simulink model "aerodynamic_model_V1_1_Coupling"  (R2025b)
settings: Solver=ode4  StartTime=0.0  StopTime=8  FixedStep=Ts  RelTol=1e-3
InitFcn:
  | % Run initial_main.m first to load Ad,As,Tq_prop,Tq_mass,...
values from neighbouring files (symbols this model uses):
  alpha_du0_v_tail_L = trim_aero_ic.v_tail_L.alpha_du0    [initial_main_V1_1.m]
  alpha_du0_v_tail_R = trim_aero_ic.v_tail_R.alpha_du0    [initial_main_V1_1.m]
  alpha_du0_wing_L = trim_aero_ic.wing_L.alpha_du0    [initial_main_V1_1.m]
  alpha_du0_wing_R = trim_aero_ic.wing_R.alpha_du0    [initial_main_V1_1.m]
  As = sys_sd.A    [initial_main_V1_1.m]
  BladePitch_deg = 34    [initial_main_V1_1.m]
  Bs = sys_sd.B    [initial_main_V1_1.m]
  Cs = sys_sd.C    [initial_main_V1_1.m]
  ctrl_delta_lim_deg = strips.delta_lim_deg    [initial_main_V1_1.m]
  ctrl_map_aileron_L = aero.wing_L.map_aileron(:)    [initial_main_V1_1.m]
  ctrl_map_aileron_R = aero.wing_R.map_aileron(:)    [initial_main_V1_1.m]
  ctrl_map_tail_L = aero.v_tail_L.map_tail(:)    [initial_main_V1_1.m]
  ctrl_map_tail_R = aero.v_tail_R.map_tail(:)    [initial_main_V1_1.m]
  Ds = sys_sd.D    [initial_main_V1_1.m]
  I_cg_b = R_sb * I_cg_m * R_sb.'    [aeroelastic.m]    (also in initial_main_V1_1.m = grav.I_cg_b)
  I_cg_b_inv = R_sb * I_cg_m_inv * R_sb.'    [aeroelastic.m]    (also in initial_main_V1_1.m = grav.I_cg_b_inv)
  m_total_kg = grav.m_total_kg    [initial_main_V1_1.m]
  n_modes = size(Phi, 2)    [aeroelastic.m]    (also in initial_main_V1_1.m = n_rigid + n_elastic)
  ones_1_tail = ones(1, size(r_cg2ac_b_v_tail_L, 2))    [initial_main_V1_1.m]
  ones_1_wing = ones(1, size(r_cg2ac_b_wing_L, 2))    [initial_main_V1_1.m]
  polar_alpha_deg = polar.alpha_deg(:).'    [initial_main_V1_1.m]
  polar_CD = polar.CD(:).'    [initial_main_V1_1.m]
  polar_CDp = polar.CDp(:).'    [initial_main_V1_1.m]
  polar_CL = polar.CL(:).'    [initial_main_V1_1.m]
  polar_CM = polar.CM(:).'    [initial_main_V1_1.m]
  r_cg2ac_b_v_tail_L = R_sb * aero.v_tail_L.r_ac_s    [initial_main_V1_1.m]
  r_cg2ac_b_v_tail_R = R_sb * aero.v_tail_R.r_ac_s    [initial_main_V1_1.m]
  r_cg2ac_b_wing_L = R_sb * aero.wing_L.r_ac_s    [initial_main_V1_1.m]
  r_cg2ac_b_wing_R = R_sb * aero.wing_R.r_ac_s    [initial_main_V1_1.m]
  r_cg2kink_b = eng.r_cg2kink_b    [initial_main_V1_1.m]
  r_cg2node_b = aeroelastic.node_arms(nodes, 'R_sb', R_sb).r_cg2node_b    [initial_main_V1_1.m]
  T_aero2W = aeroelastic.wing_aileron_to_W(strips).T    [initial_main_V1_1.m]
  T_prop2W = load_maps.T_prop2W    [initial_main_V1_1.m]
  Tq_mass = load_maps.Tq_mass    [initial_main_V1_1.m]
  trim_Attitude_rad0 = trim_default.Attitude_rad0    [initial_main_V1_1.m]
  trim_Omega_b0 = trim_default.Omega_b0    [initial_main_V1_1.m]
  trim_Position0 = trim_default.Position0    [initial_main_V1_1.m]
  trim_Velocity_b0 = trim_default.Velocity_b0    [initial_main_V1_1.m]
  Ts = 0.001    [initial_main_V1_1.m]
  U = 50    [initial_main_V1_1.m]
  v_tail_cant_rad = deg2rad(v_tail_cant_deg)    [initial_main_V1_1.m]
  W_mass_g = grav.W_mass    [initial_main_V1_1.m]
  x0_structure = trim_default.x0_structure    [initial_main_V1_1.m]
  x0_wagner_v_tail_L = trim_aero_ic.v_tail_L.x0_wagner    [initial_main_V1_1.m]
  x0_wagner_v_tail_R = trim_aero_ic.v_tail_R.x0_wagner    [initial_main_V1_1.m]
  x0_wagner_wing_L = trim_aero_ic.wing_L.x0_wagner    [initial_main_V1_1.m]
  x0_wagner_wing_R = trim_aero_ic.wing_R.x0_wagner    [initial_main_V1_1.m]
undefined symbols (not defined in the file or in its folder): Ad_v_tail_L, Ad_v_tail_R, Ad_wing_L, Ad_wing_R, Bd_v_tail_L, Bd_v_tail_R, Bd_wing_L, Bd_wing_R, c_over_2U_v_tail_L, c_over_2U_v_tail_R, c_over_2U_wing_L, c_over_2U_wing_R, Cd_v_tail_L, Cd_v_tail_R, Cd_wing_L, Cd_wing_R, Dd_v_tail_L, Dd_v_tail_R, Dd_wing_L, Dd_wing_R, G_du_v_tail_L, G_du_v_tail_R, G_du_wing_L, G_du_wing_R, polar_aileron_alpha_deg, polar_aileron_dCD, polar_aileron_dCL, polar_aileron_dCM, polar_aileron_delta_deg, polar_ruddervator_alpha_deg, polar_ruddervator_dCD, polar_ruddervator_dCL, polar_ruddervator_dCM, polar_ruddervator_delta_deg, qS_strip_v_tail_L, qS_strip_v_tail_R, qS_strip_wing_L, qS_strip_wing_R, qSc_strip_v_tail_L, qSc_strip_v_tail_R, qSc_strip_wing_L, qSc_strip_wing_R, T_m2b_v_tail_L, T_m2b_v_tail_R, T_m2b_wing_L, T_m2b_wing_R, T_m2h_v_tail_L, T_m2h_v_tail_R, T_m2h_wing_L, T_m2h_wing_R, Tq_CM_v_tail_L, Tq_CM_v_tail_R, Tq_CM_wing_L, Tq_CM_wing_R, Tq_D_v_tail_L, Tq_D_v_tail_R, Tq_D_wing_L, Tq_D_wing_R, Tq_v_tail_L, Tq_v_tail_R ... (+2)
libraries: Prop_gryo x9, matrix_library x2
(part 2 of 2)

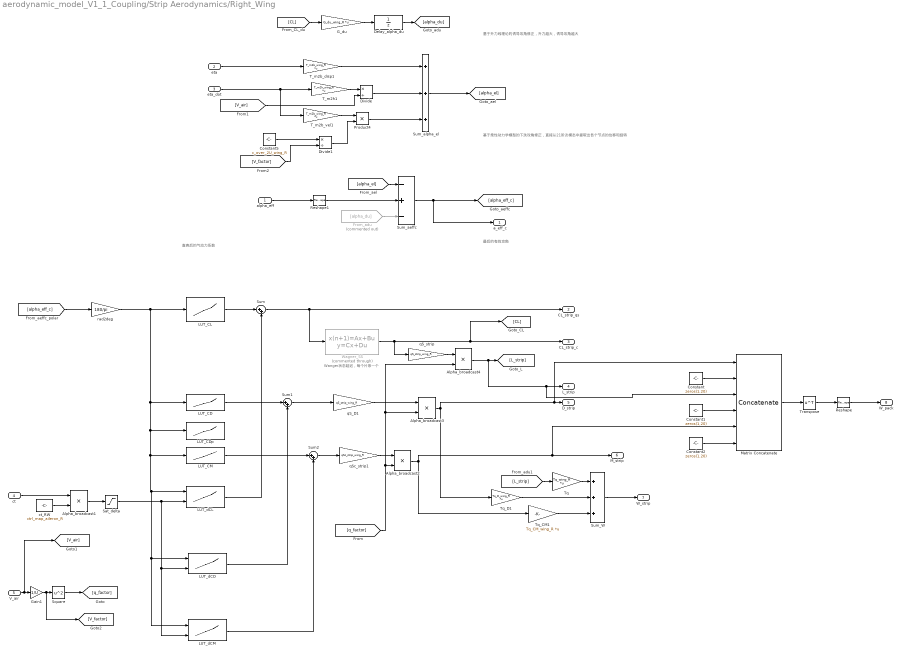
== system aerodynamic_model_V1_1_Coupling/Strip Aerodynamics/Right_Wing ==
  note: Wanger状态延迟，每个片条一个
  note: 查表后的气动力系数
  note: 最后的有效攻角
  note: 基于柔性动力学模型的下洗攻角修正，直接从21阶次模态中提取出各个节点的位移和旋转
  note: 基于升力线理论的诱导攻角修正，升力越大，诱导攻角越大
  alpha_eff : Inport
  eta : Inport  Port=2
  eta_dot : Inport  Port=3
  ct : Inport  Port=4
  V_air : Inport  Port=5
  Alpha_broadcast{1..4} (4 alike) : Product  Inputs=**
  Constant : Constant  Value=zeros(1,20)
  Constant1 : Constant  Value=zeros(1,20)
  Constant2 : Constant  Value=zeros(1,20)
  Constant5 : Constant  Value=c_over_2U_wing_R
  Delay_alpha_du : UnitDelay  InitialCondition=alpha_du0_wing_R  SampleTime=Ts  HasFrameUpgradeWarning=on
  Divide : Product  Inputs=*/
  Divide1 : Product  Inputs=*/
  From_adu : From  Commented=on  GotoTag=alpha_du
  G_du : Gain  Gain=G_du_wing_R  Multiplication=Matrix(K*u)
  Gain1 : Gain  Gain=1/U
  LUT_CD : Lookup_n-D  NumberOfTableDimensions=1  BreakpointsForDimension1=polar_alpha_deg  BreakpointsForDimension3=[5, 7]  Table=polar_CD  ExtrapMethod=Clip  InternalRulePriority=Speed  RndMeth=Simplest
  LUT_CDp : Lookup_n-D  NumberOfTableDimensions=1  BreakpointsForDimension1=polar_alpha_deg  BreakpointsForDimension3=[5, 7]  Table=polar_CDp  ExtrapMethod=Clip  InternalRulePriority=Speed  RndMeth=Simplest
  LUT_CL : Lookup_n-D  NumberOfTableDimensions=1  BreakpointsForDimension1=polar_alpha_deg  BreakpointsForDimension3=[5, 7]  Table=polar_CL  ExtrapMethod=Clip  InternalRulePriority=Speed  RndMeth=Simplest
  LUT_CM : Lookup_n-D  NumberOfTableDimensions=1  BreakpointsForDimension1=polar_alpha_deg  BreakpointsForDimension3=[5, 7]  Table=polar_CM  ExtrapMethod=Clip  InternalRulePriority=Speed  RndMeth=Simplest
  LUT_dCD : Lookup_n-D  BreakpointsForDimension1=polar_aileron_alpha_deg  BreakpointsForDimension2=polar_aileron_delta_deg  BreakpointsForDimension3=[5, 7]  Table=polar_aileron_dCD  ExtrapMethod=Clip  InternalRulePriority=Speed  RndMeth=Simplest
      settings: InputPortMap=u0,u1
  LUT_dCL : Lookup_n-D  BreakpointsForDimension1=polar_aileron_alpha_deg  BreakpointsForDimension2=polar_aileron_delta_deg  BreakpointsForDimension3=[5, 7]  Table=polar_aileron_dCL  ExtrapMethod=Clip  InternalRulePriority=Speed  RndMeth=Simplest
      settings: InputPortMap=u0,u1
  LUT_dCM : Lookup_n-D  BreakpointsForDimension1=polar_aileron_alpha_deg  BreakpointsForDimension2=polar_aileron_delta_deg  BreakpointsForDimension3=[5, 7]  Table=polar_aileron_dCM  ExtrapMethod=Clip  InternalRulePriority=Speed  RndMeth=Simplest
      settings: InputPortMap=u0,u1
  Matrix Concatenate : Concatenate  NumInputs=6  Mode=Multidimensional array  ConcatenateDimension=2
  Product4 : Product
  Reshape : Reshape
  Reshape1 : Reshape
  Sat_delta : Saturate  UpperLimit=ctrl_delta_lim_deg  LowerLimit=-ctrl_delta_lim_deg
  Square : Math  Operator=square
  Sum : Sum  Inputs=|++
  Sum1 : Sum  Inputs=|++
  Sum2 : Sum  Inputs=|++
  Sum_W : Sum  Inputs=+++
  Sum_aeffc : Sum  Inputs=-+-
  Sum_alpha_el : Sum  Inputs=+++
  T_m2b_disp1 : Gain  Gain=T_m2b_wing_R  Multiplication=Matrix(K*u)
  T_m2b_vel1 : Gain  Gain=T_m2b_wing_R  Multiplication=Matrix(K*u)
  T_m2h1 : Gain  Gain=T_m2h_wing_R  Multiplication=Matrix(K*u)
  Tq : Gain  Gain=Tq_wing_R  Multiplication=Matrix(K*u)
  Tq_CM1 : Gain  Gain=Tq_CM_wing_R  Multiplication=Matrix(K*u)
  Tq_D1 : Gain  Gain=Tq_D_wing_R  Multiplication=Matrix(K*u)
  Transpose : Math  Operator=transpose
  Wagner_SS : DiscreteStateSpace  Commented=through  A=Ad_wing_R  B=Bd_wing_R  C=Cd_wing_R  D=Dd_wing_R  InitialCondition=x0_wagner_wing_R  SampleTime=Ts
  ct_RW : Constant  Value=ctrl_map_aileron_R
  qS_D1 : Gain  Gain=qS_strip_wing_R
  qS_strip : Gain  Gain=qS_strip_wing_R
  qSc_strip1 : Gain  Gain=qSc_strip_wing_R
  rad2deg : Gain  Gain=180/pi
  a_eff_c : Outport
  CL_strip_qs : Outport  Port=2
  CL_strip_c : Outport  Port=3
  L_strip : Outport  Port=4
  D_strip : Outport  Port=5
  M_strip : Outport  Port=6
  W_strip : Outport  Port=7
  W_pack : Outport  Port=8
  wires:
  Sat_delta/1 -> LUT_dCL/2, LUT_dCD/2, LUT_dCM/2
  LUT_dCM/1 -> Sum2/2
  LUT_CM/1 -> Sum2/1
  LUT_dCD/1 -> Sum1/2
  LUT_CD/1 -> Sum1/1
  LUT_dCL/1 -> Sum/2
  LUT_CL/1 -> Sum/1
  Alpha_broadcast1/1 -> Sat_delta/1
  ct_RW/1 -> Alpha_broadcast1/2
  ct/1 -> Alpha_broadcast1/1
  alpha_eff/1 -> Reshape1/1
  Sum_W/1 -> W_strip/1
  Tq_CM1/1 -> Sum_W/3
  Tq_D1/1 -> Sum_W/2
  Tq/1 -> Sum_W/1
  [L_strip] -> Tq/1
  From_adu/1 -> Sum_aeffc/3
  [alpha_el] -> Sum_aeffc/1
  [CL] -> G_du/1
  Sum2/1 -> qSc_strip1/1
  Sum1/1 -> qS_D1/1
  [alpha_eff_c] -> rad2deg/1
  Sum_aeffc/1 -> [alpha_eff_c], a_eff_c/1
  Sum_alpha_el/1 -> [alpha_el]
  G_du/1 -> Delay_alpha_du/1
  Sum/1 -> Wagner_SS/1, CL_strip_qs/1
  Delay_alpha_du/1 -> [alpha_du]
  Wagner_SS/1 -> qS_strip/1, [CL], CL_strip_c/1
  rad2deg/1 -> LUT_CL/1, LUT_CM/1, LUT_dCL/1, LUT_dCD/1, LUT_dCM/1, LUT_CDp/1, LUT_CD/1
  Alpha_broadcast4/1 -> Matrix Concatenate/3, L_strip/1, [L_strip]
  Transpose/1 -> Reshape/1
  Reshape/1 -> W_pack/1
  Alpha_broadcast2/1 -> Tq_CM1/1, Matrix Concatenate/5, M_strip/1
  Alpha_broadcast3/1 -> Matrix Concatenate/1, D_strip/1, Tq_D1/1
  Matrix Concatenate/1 -> Transpose/1
  Constant/1 -> Matrix Concatenate/2
  Constant1/1 -> Matrix Concatenate/4
  Constant2/1 -> Matrix Concatenate/6
  Reshape1/1 -> Sum_aeffc/2
  V_air/1 -> [V_air], Gain1/1
  Square/1 -> [q_factor]
  [q_factor] -> Alpha_broadcast4/2, Alpha_broadcast3/2, Alpha_broadcast2/2
  qSc_strip1/1 -> Alpha_broadcast2/1
  qS_D1/1 -> Alpha_broadcast3/1
  qS_strip/1 -> Alpha_broadcast4/1
  [V_factor] -> Divide1/2
  Divide1/1 -> Product4/2
  T_m2h1/1 -> Divide/1
  Product4/1 -> Sum_alpha_el/3
  T_m2b_vel1/1 -> Product4/1
  T_m2b_disp1/1 -> Sum_alpha_el/1
  eta_dot/1 -> T_m2b_vel1/1, T_m2h1/1
  eta/1 -> T_m2b_disp1/1
  Divide/1 -> Sum_alpha_el/2
  Constant5/1 -> Divide1/1
  [V_air] -> Divide/2
  Gain1/1 -> [V_factor], Square/1

== matlab function aerodynamic_model_V1_1_Coupling/Strip Aerodynamics/Local_Alphas/MATLAB Function3 ==
  data: V input; alpha output; beta output
function [alpha, beta] = fcn(V)
[alpha, beta] = strip_aero_angles(V);
end

== matlab function aerodynamic_model_V1_1_Coupling/Strip Aerodynamics/Local_Alphas/MATLAB Function1 ==
  data: V input; alpha output; beta output
function [alpha, beta] = fcn(V)
[alpha, beta] = strip_aero_angles(V);
end

== matlab function aerodynamic_model_V1_1_Coupling/Strip Aerodynamics/Local_Alphas/MATLAB Function2 ==
  data: V input; alpha output; beta output
function [alpha, beta] = fcn(V)
[alpha, beta] = strip_aero_angles(V);
end

== matlab function aerodynamic_model_V1_1_Coupling/Strip Aerodynamics/Local_Alphas/MATLAB Function4 ==
  data: V input; alpha output; beta output
function [alpha, beta] = fcn(V)
[alpha, beta] = strip_aero_angles(V);
end

== matlab function aerodynamic_model_V1_1_Coupling/Strip Aerodynamics/Local_Alphas/MATLAB Function ==
  data: omega input; Omega_skew output
function Omega_skew = fcn(omega)
p=omega(1);
q=omega(2);
r=omega(3);

Omega_skew =  [0 -r q;r 0 -p;-q p 0];

== matlab function aerodynamic_model_V1_1_Coupling/Flexible Aircraft Dynamics/MATLAB Function2 ==
  data: F input; F_cg output; M input; r input; M_cg output
function [F_cg, M_cg] = wrench_to_cg(F, M, r) %#codegen
%WRENCH_TO_CG  节点力/力矩合到质心
%
%  [F_cg, M_cg] = wrench_to_cg(F, M, r)
%
%  F, M, r  3×n  每列一个节点，必须同一坐标系
%            r 用 r_cg2node_m（结构）或 r_cg2node_b（机体）
%  F_cg     3×1  Σ F
%  M_cg     3×1  Σ (r × F + M)
%
%  不要把 6 维扳手整段叉乘。力只求和；力矩才是 r×F 再加节点力矩。

    F_cg = sum(F, 2);
    M_cg = sum(cross3n(r, F) + M, 2);
end

== matlab function aerodynamic_model_V1_1_Coupling/Flexible Aircraft Dynamics/MATLAB Function3 ==
  data: p input; phi_dot output; q input; r input; phi input; theta input; theta_dot output; psi_dot output
function [phi_dot, theta_dot, psi_dot] = euler_kinematics(p, q, r, phi, theta)
    % 输入：
    %   p, q, r  - 体轴角速度 (rad/s)
    %   phi      - 滚转角 (rad)
    %   theta    - 俯仰角 (rad)
    % 输出：
    %   phi_dot, theta_dot, psi_dot - 欧拉角变化率 (rad/s)
    
    % 保护：防止 theta = ±90° 时除零（万向节锁）
    cos_theta = cos(theta);
    if abs(cos_theta) < 1e-6
        cos_theta = sign(cos_theta) * 1e-6;  % 保留符号，避免符号跳变
    end
    
    tan_theta = sin(theta) / cos_theta;
    
    % 运动学矩阵
    phi_dot   = p + q * sin(phi) * tan_theta + r * cos(phi) * tan_theta;
    theta_dot = q * cos(phi) - r * sin(phi);
    psi_dot   = (q * sin(phi) + r * cos(phi)) / cos_theta;
end
